simulink model "HalfQuadOL"  (R2025b)
settings: Solver=ode1  StartTime=0.0  StopTime=40  FixedStep=0.002  RelTol=1e-3  EnableMultiTasking=on
PreLoadFcn:
  | % quanser_aero_pd_design;
values from neighbouring files (symbols this model uses):
  Dm = 0.0071    [QuanserData.m]
  Dp = 0.0071    [QuanserData.m]
  Dt = 0.158    [QuanserData.m]
  g = 9.81    [QuanserData.m]
  Jeq = Jm+Jh+Jp    (= 1.120304e-05)    [QuanserData.m]
  Jp = 2.15e-2    (= 0.0215)    [QuanserData.m]
  k1 = 1.2e-5    (= 1.2e-05)    [QuanserData.m]
  k2 = 3.54e-9    (= 3.54e-09)    [QuanserData.m]
  k3 = 0    [QuanserData.m]
  k4 = 6.23e-7    (= 6.23e-07)    [QuanserData.m]
  km = 0.042    [QuanserData.m]
  Mb = 1.15    [QuanserData.m]
  Rm = 8.4    [QuanserData.m]
undefined symbols (not defined in the file or in its folder): HIL
libraries: quarc_library x8
settings Model: ExtModeTrigDuration=1000000  Creator=MLevis  LastModifiedBy=pakaw
settings SolverCC: AlgebraicLoopSolver=TrustRegion  PositivePriorityOrder=on  AutoInsertRateTranBlk=on
settings DataIOCC: LimitDataPoints=on  SaveFormat=Array  ReturnWorkspaceOutputs=off
settings DebuggingCC: SolverPrmCheckMsg=warning  UnconnectedInputMsg=warning  UnconnectedOutputMsg=warning  UnconnectedLineMsg=warning  SFUnexpectedBacktrackingDiag=warning  SFNoUnconditionalDefaultTransitionDiag=warning  SFExecutionAtInitializationDiag=none  ArithmeticOperatorsInVariantConditions=warning
settings ModelReferenceCC: EnableRefExpFcnMdlSchedulingChecks=on  PropagateSignalLabelsOutOfModel=off
settings SFSimCC: SimUseLocalCustomCode=off  CustomCodeUndefinedFunction=UseInterfaceOnly
settings RTWCC: SystemTargetFile=quarc_win64.tlc  TemplateMakefile=quarc_default_tmf  RTWUseLocalCustomCode=off  Toolchain=QUARC win64 | nmake (64-bit Windows)  BuildConfiguration=Faster Runs  GPUComputeCapability=3.5  Description=QUARC Win64 Target Using Toolchain
settings CodeAppCC: StateflowObjectComments=on
settings STFCustomTargetCC: SystemTargetFile=quarc_win64.tlc  UseToolchainInfoCompliant=on
settings GRTTargetCC: ExtMode=on  ExtModeMexFile=quarc_comm  TargetLangStandard=C89/C90 (ANSI)  ParMdlRefBuildCompliant=off  CompOptLevelCompliant=off  CombineOutputUpdateFcns=off  MatFileLogging=off  CPPClassGenCompliant=off  GRTInterface=on
settings ConfigComp: CovMetricSettings=dw  CovSaveCumulativeToWorkspaceVar=on  CovSaveSingleToWorkspaceVar=on  CovExternalEMLEnable=off  CovSFcnEnable=off

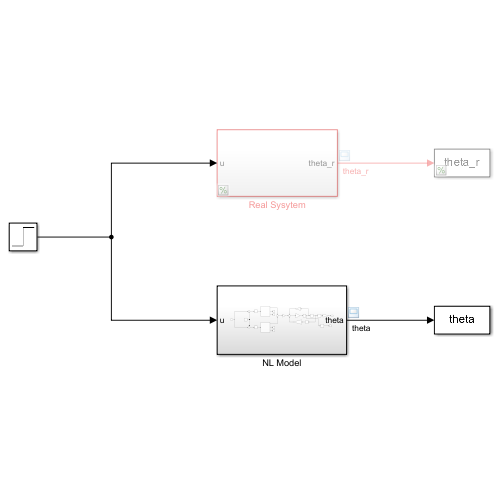
[thumbnail: Simulink's stored preview of the top-level diagram]
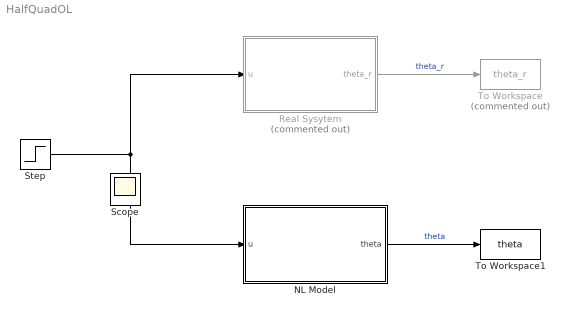
== system HalfQuadOL ==
  NL Model : Subsystem
  Real Sysytem : Subsystem  Commented=on
  Step : Step  Time=2  After=10  SampleTime=0
  To Workspace : ToWorkspace  Commented=on  VariableName=theta_r  SaveFormat=Structure With Time  SampleTime=-1
  To Workspace1 : ToWorkspace  VariableName=theta  SaveFormat=Structure With Time  SampleTime=-1
  Scope : Scope
      settings: ActiveDisplayYMinimum=-3.10109  ActiveDisplayYMaximum=27.90978
  wires:
  Step/1 -> NL Model/1(u), Real Sysytem/1(u)
  Real Sysytem/1(theta_r) -> To Workspace/1  "theta_r"
  NL Model/1(theta) -> To Workspace1/1  "theta"

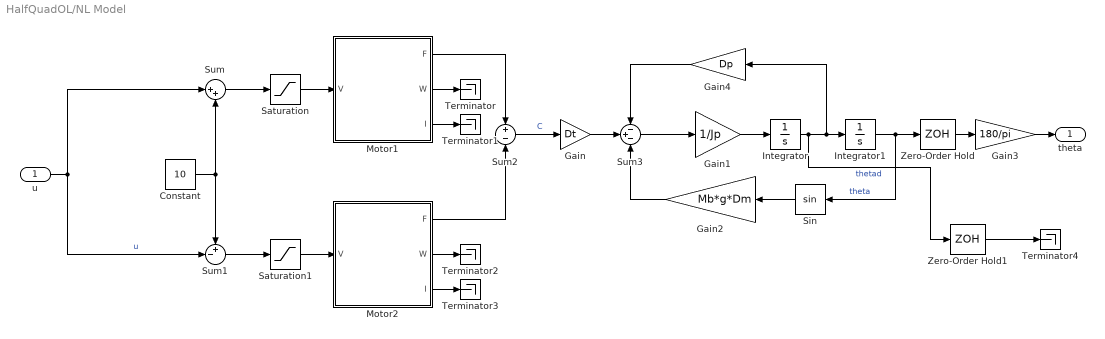
== system HalfQuadOL/NL Model ==
  u : Inport
  Constant : Constant  Value=10
  Gain : Gain  Gain=Dt
  Gain1 : Gain  Gain=1/Jp
  Gain2 : Gain  Gain=Mb*g*Dm
  Gain3 : Gain  Gain=180/pi
  Gain4 : Gain  Gain=Dp
  Integrator : Integrator
  Integrator1 : Integrator
  Motor1 : Subsystem
  Motor2 : Subsystem
  Saturation : Saturate  UpperLimit=24  LowerLimit=-24
  Saturation1 : Saturate  UpperLimit=24  LowerLimit=-24
  Sin : Trigonometry
  Sum : Sum  Inputs=|++
  Sum1 : Sum  Inputs=+-|
  Sum2 : Sum  Inputs=+-
  Sum3 : Sum  Inputs=-+-
  Terminator{,1..4} (5 alike) : Terminator
  Zero-Order Hold : ZeroOrderHold  SampleTime=2e-3
  Zero-Order Hold1 : ZeroOrderHold  SampleTime=2e-3
  theta : Outport  VectorParamsAs1DForOutWhenUnconnected=off
  wires:
  Sum2/1 -> Gain/1  "C"
  u/1 -> Sum/1, Sum1/2  "u"
  Motor1/2(W) -> Terminator/1
  Constant/1 -> Sum1/1, Sum/2
  Motor1/3(I) -> Terminator1/1
  Motor2/3(I) -> Terminator3/1
  Integrator/1 -> Zero-Order Hold1/1, Gain4/1, Integrator1/1  "thetad"
  Integrator1/1 -> Zero-Order Hold/1, Sin/1  "theta"
  Motor2/2(W) -> Terminator2/1
  Sum/1 -> Saturation/1
  Sum3/1 -> Gain1/1
  Gain4/1 -> Sum3/1
  Gain/1 -> Sum3/2
  Sum1/1 -> Saturation1/1
  Motor2/1(F) -> Sum2/2
  Gain1/1 -> Integrator/1
  Motor1/1(F) -> Sum2/1
  Sin/1 -> Gain2/1
  Gain2/1 -> Sum3/3
  Saturation/1 -> Motor1/1(V)
  Saturation1/1 -> Motor2/1(V)
  Zero-Order Hold/1 -> Gain3/1
  Zero-Order Hold1/1 -> Terminator4/1
  Gain3/1 -> theta/1

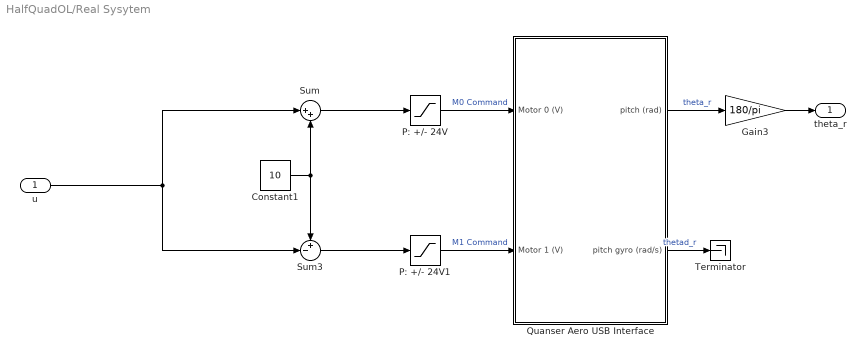
== system HalfQuadOL/Real Sysytem ==
  u : Inport
  Constant1 : Constant  Value=10
  Gain3 : Gain  Gain=180/pi
  P: +/- 24V : Saturate  UpperLimit=24  LowerLimit=-24
  P: +/- 24V1 : Saturate  UpperLimit=24  LowerLimit=-24
  Quanser Aero USB Interface : Subsystem
  Sum : Sum  Inputs=|++
  Sum3 : Sum  Inputs=+-|
  Terminator : Terminator
  theta_r : Outport  VectorParamsAs1DForOutWhenUnconnected=off
  wires:
  Constant1/1 -> Sum3/1, Sum/2
  u/1 -> Sum/1, Sum3/2
  P: +/- 24V1/1 -> Quanser Aero USB Interface/2(Motor 1 (V))  "M1 Command"
  Sum/1 -> P: +/- 24V/1
  Sum3/1 -> P: +/- 24V1/1
  Quanser Aero USB Interface/1(pitch (rad)) -> Gain3/1  "theta_r"
  P: +/- 24V/1 -> Quanser Aero USB Interface/1(Motor 0 (V))  "M0 Command"
  Quanser Aero USB Interface/2(pitch gyro (rad/s)) -> Terminator/1  "thetad_r"
  Gain3/1 -> theta_r/1

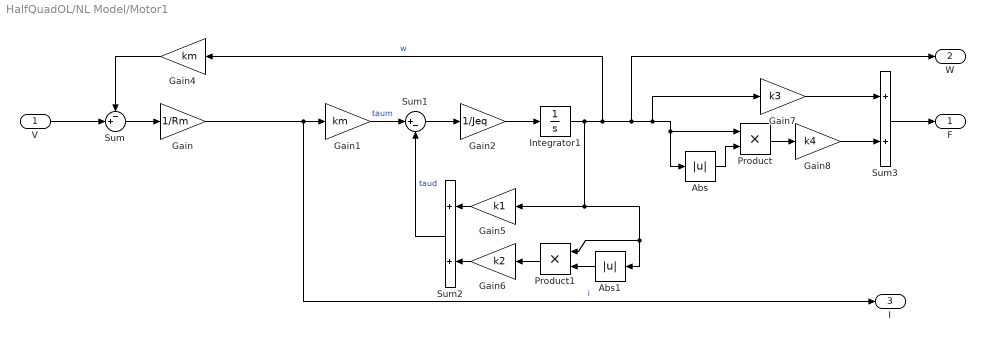
== system HalfQuadOL/NL Model/Motor1 ==
  V : Inport
  Abs : Abs  SaturateOnIntegerOverflow=off
  Abs1 : Abs  SaturateOnIntegerOverflow=off
  Gain : Gain  Gain=1/Rm
  Gain1 : Gain  Gain=km
  Gain2 : Gain  Gain=1/Jeq
  Gain4 : Gain  Gain=km
  Gain5 : Gain  Gain=k1
  Gain6 : Gain  Gain=k2
  Gain7 : Gain  Gain=k3
  Gain8 : Gain  Gain=k4
  Integrator1 : Integrator
  Product : Product
  Product1 : Product
  Sum : Sum  Inputs=-+|
  Sum1 : Sum  Inputs=|+-
  Sum2 : Sum
  Sum3 : Sum
  F : Outport  VectorParamsAs1DForOutWhenUnconnected=off
  W : Outport  Port=2  VectorParamsAs1DForOutWhenUnconnected=off
  I : Outport  Port=3  VectorParamsAs1DForOutWhenUnconnected=off
  wires:
  Gain5/1 -> Sum2/1
  Sum3/1 -> F/1
  Gain8/1 -> Sum3/2
  Product1/1 -> Gain6/1
  Gain4/1 -> Sum/1
  Product/1 -> Gain8/1
  Sum1/1 -> Gain2/1
  Gain6/1 -> Sum2/2
  Sum2/1 -> Sum1/2  "taud"
  Gain/1 -> I/1, Gain1/1  "i"
  Sum/1 -> Gain/1
  Gain7/1 -> Sum3/1
  Integrator1/1 -> Abs1/1, Product1/1, Gain5/1, W/1, Abs/1, Product/1, Gain7/1, Gain4/1  "w"
  Gain1/1 -> Sum1/1  "taum"
  Gain2/1 -> Integrator1/1
  V/1 -> Sum/2
  Abs/1 -> Product/2
  Abs1/1 -> Product1/2

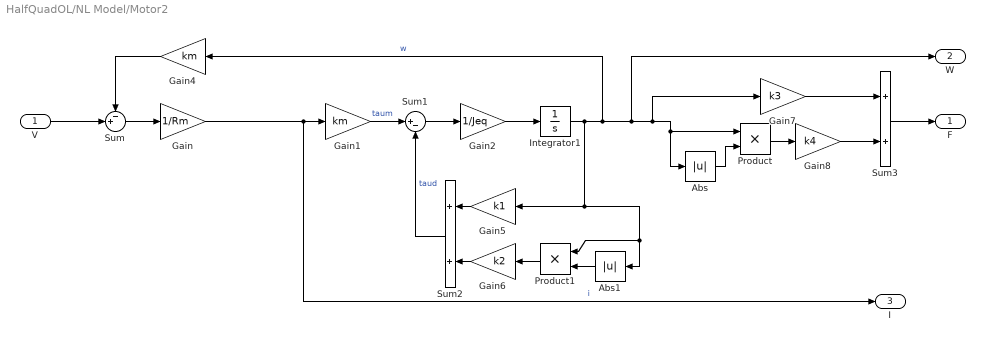
== system HalfQuadOL/NL Model/Motor2 ==
  V : Inport
  Abs : Abs  SaturateOnIntegerOverflow=off
  Abs1 : Abs  SaturateOnIntegerOverflow=off
  Gain : Gain  Gain=1/Rm
  Gain1 : Gain  Gain=km
  Gain2 : Gain  Gain=1/Jeq
  Gain4 : Gain  Gain=km
  Gain5 : Gain  Gain=k1
  Gain6 : Gain  Gain=k2
  Gain7 : Gain  Gain=k3
  Gain8 : Gain  Gain=k4
  Integrator1 : Integrator
  Product : Product
  Product1 : Product
  Sum : Sum  Inputs=-+|
  Sum1 : Sum  Inputs=|+-
  Sum2 : Sum
  Sum3 : Sum
  F : Outport  VectorParamsAs1DForOutWhenUnconnected=off
  W : Outport  Port=2  VectorParamsAs1DForOutWhenUnconnected=off
  I : Outport  Port=3  VectorParamsAs1DForOutWhenUnconnected=off
  wires:
  Abs1/1 -> Product1/2
  Abs/1 -> Product/2
  V/1 -> Sum/2
  Gain2/1 -> Integrator1/1
  Gain1/1 -> Sum1/1  "taum"
  Integrator1/1 -> Gain4/1, Gain7/1, Product/1, Abs/1, W/1, Gain5/1, Product1/1, Abs1/1  "w"
  Gain7/1 -> Sum3/1
  Sum/1 -> Gain/1
  Gain/1 -> Gain1/1, I/1  "i"
  Sum2/1 -> Sum1/2  "taud"
  Gain6/1 -> Sum2/2
  Sum1/1 -> Gain2/1
  Product/1 -> Gain8/1
  Gain4/1 -> Sum/1
  Product1/1 -> Gain6/1
  Gain8/1 -> Sum3/2
  Sum3/1 -> F/1
  Gain5/1 -> Sum2/1

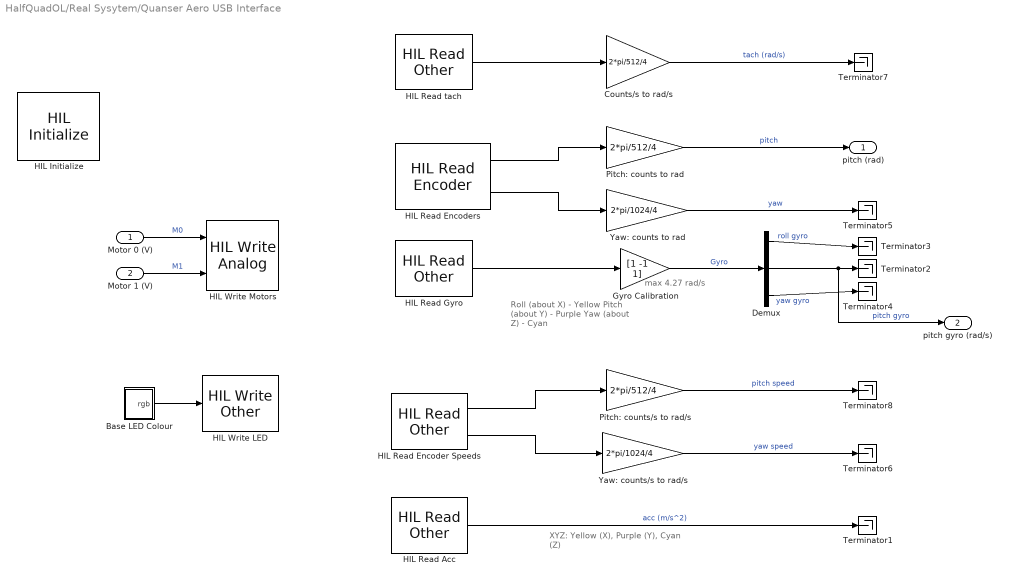
== system HalfQuadOL/Real Sysytem/Quanser Aero USB Interface ==
  note: max 4.27 rad/s
  note: Roll (about X) - Yellow
      | Pitch (about Y) - Purple
      | Yaw (about Z) - Cyan
  note: XYZ:
      | Yellow (X), Purple (Y), Cyan (Z)
  Motor 0 (V) : Inport
  Motor 1 (V) : Inport  Port=2
  Base LED Colour : Subsystem  mask(Color Constant){color=[0 0 1]}
      mask help: Outputs a constant RGB color value.
      mask init:
      | rgb = get_param(gcbh, 'color');
      | if numel(color) ~= 3
      |     rgb = [0 0 0];
      | end
      | set_param(gcbh, 'MaskDisplay', ['patch([-0.02 -0.02 1.02 1.02], [-0.02 1.02 1.02 -0.02], ', rgb, ');']);
      settings: OpenFcn=color_constant_properties('CurrentBlock', gcbh);
      mask Help: web(qc_get_block_help_path(gcb), '-helpbrowser');
      mask Display: patch([-0.02 -0.02 1.02 1.02], [-0.02 1.02 1.02 -0.02], [0 0 1]);
  Counts/s to rad/s : Gain  Gain=2*pi/512/4
  Demux : Demux  Outputs=3
  Gyro Calibration : Gain  Gain=[1 -1 1]
  HIL Initialize : quarc_library/Data Acquisition/Generic/Configuration/HIL Initialize  Priority=-99  object_name=HIL-1  board_type=quanser_aero_usb  board_number=0  board_options=""  exclusive=off  active=off  hardware_clocks=[0]  clock_modes=[]  initial_clock_frequencies=[]  set_clock_params_at_start=off  set_clock_params_at_switch_in=off  set_clock_frequencies_at_start=off  set_clock_frequencies_at_switch_in=off  analog_input_channels=[0:1]  analog_input_configurations=[]  analog_input_maximums=3  analog_input_minimums=-3  set_analog_input_params_at_start=off  set_analog_input_params_at_switch_in=off  analog_output_channels=[0:1]  analog_output_maximums=24  analog_output_minimums=-24  initial_analog_outputs=[0]  final_analog_outputs=[0]  watchdog_analog_outputs=[0]  set_analog_output_params_at_start=off  set_analog_output_params_at_switch_in=off  set_analog_outputs_at_start=on  set_analog_outputs_at_switch_in=off  set_analog_outputs_at_terminate=on  set_analog_outputs_at_switch_out=off  set_analog_outputs_on_watchdog=on  digital_input_channels=[]  digital_output_channels=[0:1]  digital_output_configuration=[]  initial_digital_outputs=[1]  final_digital_outputs=[0]  watchdog_digital_outputs=[0]  set_digital_output_params_at_start=off  set_digital_output_params_at_switch_in=off  set_digital_outputs_at_start=on  set_digital_outputs_at_switch_in=off  set_digital_outputs_at_terminate=on  set_digital_outputs_at_switch_out=off  set_digital_outputs_on_watchdog=on  encoder_channels=[0:3]  quadrature=[4]  encoder_filter_frequency=[]  initial_encoder_counts=[0]  set_encoder_params_at_start=off  set_encoder_params_at_switch_in=off  set_encoder_counts_at_start=on  set_encoder_counts_at_switch_in=off  pwm_channels=[]  pwm_modes=[]  pwm_frequency=[]  pwm_configuration=[]  pwm_alignment=[]  pwm_polarity=[]  pwm_leading_deadband=[]  pwm_trailing_deadband=[]  initial_pwm_outputs=[]  final_pwm_outputs=[]  watchdog_pwm_outputs=[]  set_pwm_params_at_start=off  set_pwm_params_at_switch_in=off  set_pwm_outputs_at_start=off  set_pwm_outputs_at_switch_in=off  set_pwm_outputs_at_terminate=off  set_pwm_outputs_at_switch_out=off  set_pwm_outputs_on_watchdog=off  other_output_channels=[11000:11002]  initial_other_outputs=[0 1 0]  final_other_outputs=[1 0 0]  watchdog_other_outputs=[0 0 1]  set_other_outputs_at_start=on  set_other_outputs_at_switch_in=off  set_other_outputs_at_terminate=on  set_other_outputs_at_switch_out=off  set_other_outputs_on_watchdog=on
  HIL Read Acc : quarc_library/Data Acquisition/Generic/Immediate I//O/HIL Read Other  object_name=HIL-1  channels=[4000:4002]  sample_time=qc_get_step_size  active=on  vector_output=on
      settings: AttributesFormatString=(%<object_name>)  SourceProductName=QUARC Targets
  HIL Read Encoder Speeds : quarc_library/Data Acquisition/Generic/Immediate I//O/HIL Read Other  object_name=HIL-1  channels=[14002:14003]  sample_time=qc_get_step_size  active=on  vector_output=off
      settings: AttributesFormatString=(%<object_name>)  SourceProductName=QUARC Targets
  HIL Read Encoders : quarc_library/Data Acquisition/Generic/Immediate I//O/HIL Read Encoder  object_name=HIL-1  channels=[2:3]  sample_time=qc_get_step_size  active=on  vector_output=off  data_type_mode=Inherit via back propagation  data_type=double
  HIL Read Gyro : quarc_library/Data Acquisition/Generic/Immediate I//O/HIL Read Other  object_name=HIL-1  channels=[3000:3002]  sample_time=qc_get_step_size  active=on  vector_output=on
      settings: AttributesFormatString=(%<object_name>)  SourceProductName=QUARC Targets
  HIL Read tach : quarc_library/Data Acquisition/Generic/Immediate I//O/HIL Read Other  object_name=HIL-1  channels=[14000:14001]  sample_time=qc_get_step_size  active=on  vector_output=on
      settings: AttributesFormatString=(%<object_name>)  SourceProductName=QUARC Targets
  HIL Write LED : quarc_library/Data Acquisition/Generic/Immediate I//O/HIL Write Other  object_name=HIL-1  channels=[11000:11002]  sample_time=-1  active=off  vector_input=on
      settings: AttributesFormatString=(%<object_name>)  SourceProductName=QUARC Targets
  HIL Write Motors : quarc_library/Data Acquisition/Generic/Immediate I//O/HIL Write Analog  object_name=HIL-1  channels=[0:1]  sample_time=-1  active=off  vector_input=off
  Pitch: counts to rad : Gain  Gain=2*pi/512/4
  Pitch: counts/s to rad/s : Gain  Gain=2*pi/512/4
  Terminator{1..8} (8 alike) : Terminator
  Yaw: counts to rad : Gain  Gain=2*pi/1024/4
  Yaw: counts/s to rad/s : Gain  Gain=2*pi/1024/4
  pitch (rad) : Outport  VectorParamsAs1DForOutWhenUnconnected=off
  pitch gyro (rad/s) : Outport  Port=2  VectorParamsAs1DForOutWhenUnconnected=off
  wires:
  Motor 1 (V)/1 -> HIL Write Motors/2  "M1"
  HIL Read Encoders/2 -> Yaw: counts to rad/1
  HIL Read Encoders/1 -> Pitch: counts to rad/1
  Motor 0 (V)/1 -> HIL Write Motors/1  "M0"
  Pitch: counts to rad/1 -> pitch (rad)/1  "pitch"
  Yaw: counts to rad/1 -> Terminator5/1  "yaw"
  Base LED Colour/1(rgb) -> HIL Write LED/1
  Gyro Calibration/1 -> Demux/1  "Gyro"
  HIL Read Gyro/1 -> Gyro Calibration/1
  HIL Read Acc/1 -> Terminator1/1  "acc (m/s^2)"
  Counts/s to rad/s/1 -> Terminator7/1  "tach (rad/s)"
  HIL Read tach/1 -> Counts/s to rad/s/1
  Pitch: counts/s to rad/s/1 -> Terminator8/1  "pitch speed"
  HIL Read Encoder Speeds/2 -> Yaw: counts/s to rad/s/1
  HIL Read Encoder Speeds/1 -> Pitch: counts/s to rad/s/1
  Yaw: counts/s to rad/s/1 -> Terminator6/1  "yaw speed"
  Demux/1 -> Terminator3/1  "roll gyro"
  Demux/3 -> Terminator4/1  "yaw gyro"
  Demux/2 -> pitch gyro (rad/s)/1, Terminator2/1  "pitch gyro"

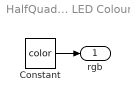
== system HalfQuadOL/Real Sysytem/Quanser Aero USB Interface/Base LED Colour ==
  Constant : Constant  Value=color
  rgb : Outport  VectorParamsAs1DForOutWhenUnconnected=off
  wires:
  Constant/1 -> rgb/1
